simulink model "can2_mcu_power_unpack"  (R2026b)
settings: Solver=VariableStepAuto
libraries: simulink x1, svdutilitieslib x1
settings Model: Creator=aomar  LastModifiedBy=aomar

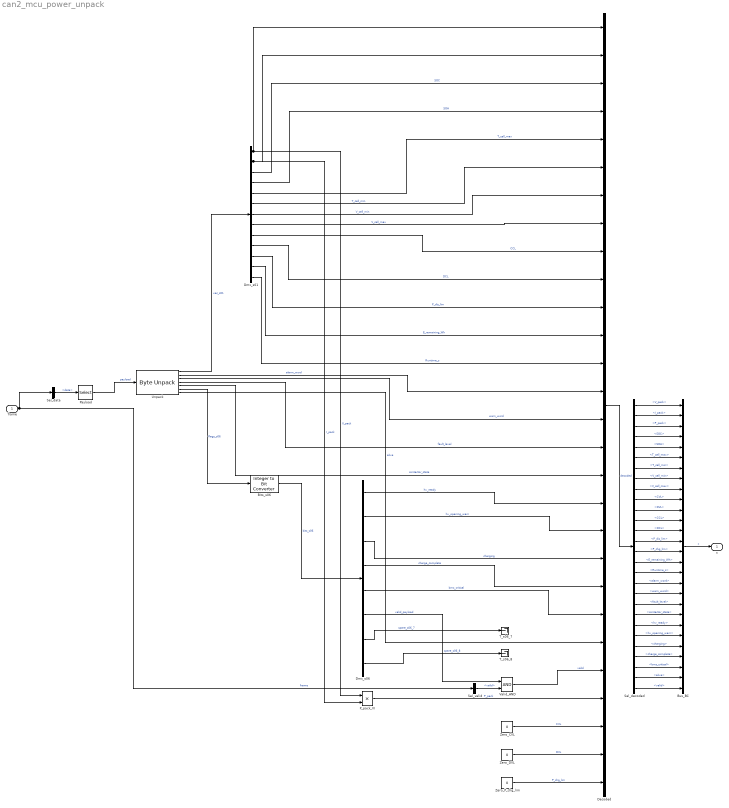
== system can2_mcu_power_unpack ==
  frame : Inport  OutDataTypeStr=Bus: Bus_CanFrame64
  Bits_s06 : simulink/Logic and Bit Operations/Integer to Bit Converter  nbits=8  signedInputValues=Unsigned  bitOrder=LSB first  outDtype=boolean
      settings: LibrarySourceBlock=|
      | commutil2/Integer to Bit
      | Converter
  Bus_BC : BusCreator  Inputs=28  OutDataTypeStr=Bus: Bus_BmsStatus  NonVirtualBus=on
      settings: InheritFromInputs=off
  Decoded : BusCreator  Inputs=28
  Dmx_s01 : Demux  Outputs=13
  Dmx_s06 : Demux  Outputs=8
  P_pack_VI : Product
  Payload : Selector  InputPortWidth=64  IndexOptions=Index vector (dialog)  Indices=1:64  OutputSizes=1
  Sel_data : BusSelector  OutputSignals=data
  Sel_decoded : BusSelector  OutputSignals=V_pack,I_pack,P_pack,SOC,SOH,T_cell_max,T_cell_min,V_cell_min,V_cell_max,CVL,DVL,CCL,DCL,P_dis_lim,P_chg_lim,E_remaining_Wh,Runtime_s,alarm_word,warn_word,fault_level,contactor_state,hv_ready,hv_opening_warn,charging,charge_complete,bms_critical,alive,valid
  Sel_valid : BusSelector  OutputSignals=valid
  T_s06_7 : Terminator
  T_s06_8 : Terminator
  Unpack : svdutilitieslib/Byte Unpack  dimensions={13,1,1,1,1,1,1}  datatypes={'single','uint32','uint32','uint8','uint8','uint8','uint8'}  byteAlign=1  blockPlatform=arduinoert
      settings: LibrarySourceBlock=mcblib/Signal Management/Byte Unpack
  Valid_AND : Logic  AllPortsSameDT=off  OutDataTypeStr=boolean
  Zero_CVL : Constant  Value=0  OutDataTypeStr=single  SampleTime=-1
  Zero_DVL : Constant  Value=0  OutDataTypeStr=single  SampleTime=-1
  Zero_P_chg_lim : Constant  Value=0  OutDataTypeStr=single  SampleTime=-1
  x : Outport  OutDataTypeStr=Bus: Bus_BmsStatus
  wires:
  frame/1 -> Sel_valid/1, Sel_data/1  "frame"
  Sel_data/1 -> Payload/1  "<data>"
  Payload/1 -> Unpack/1  "payload"
  Unpack/1 -> Dmx_s01/1  "vec_s01"
  Unpack/2 -> Decoded/14  "alarm_word"
  Unpack/3 -> Decoded/15  "warn_word"
  Unpack/4 -> Decoded/16  "fault_level"
  Unpack/5 -> Decoded/17  "contactor_state"
  Unpack/6 -> Bits_s06/1  "flags_s06"
  Unpack/7 -> Decoded/23  "alive"
  Dmx_s01/1 -> P_pack_VI/1, Decoded/1  "V_pack"
  Dmx_s01/2 -> P_pack_VI/2, Decoded/2  "I_pack"
  Dmx_s01/3 -> Decoded/3  "SOC"
  Dmx_s01/4 -> Decoded/4  "SOH"
  Dmx_s01/5 -> Decoded/5  "T_cell_max"
  Dmx_s01/6 -> Decoded/6  "T_cell_min"
  Dmx_s01/7 -> Decoded/7  "V_cell_min"
  Dmx_s01/8 -> Decoded/8  "V_cell_max"
  Dmx_s01/9 -> Decoded/9  "CCL"
  Dmx_s01/10 -> Decoded/10  "DCL"
  Dmx_s01/11 -> Decoded/11  "P_dis_lim"
  Dmx_s01/12 -> Decoded/12  "E_remaining_Wh"
  Dmx_s01/13 -> Decoded/13  "Runtime_s"
  Bits_s06/1 -> Dmx_s06/1  "bits_s06"
  Dmx_s06/1 -> Decoded/18  "hv_ready"
  Dmx_s06/2 -> Decoded/19  "hv_opening_warn"
  Dmx_s06/3 -> Decoded/20  "charging"
  Dmx_s06/4 -> Decoded/21  "charge_complete"
  Dmx_s06/5 -> Decoded/22  "bms_critical"
  Dmx_s06/6 -> Valid_AND/1  "valid_payload"
  Dmx_s06/7 -> T_s06_7/1  "spare_s06_7"
  Dmx_s06/8 -> T_s06_8/1  "spare_s06_8"
  P_pack_VI/1 -> Decoded/25  "P_pack"
  Sel_valid/1 -> Valid_AND/2  "<valid>"
  Valid_AND/1 -> Decoded/24  "valid"
  Zero_CVL/1 -> Decoded/26  "CVL"
  Zero_DVL/1 -> Decoded/27  "DVL"
  Zero_P_chg_lim/1 -> Decoded/28  "P_chg_lim"
  Decoded/1 -> Sel_decoded/1  "decoded"
  Sel_decoded/1 -> Bus_BC/1  "<V_pack>"
  Sel_decoded/2 -> Bus_BC/2  "<I_pack>"
  Sel_decoded/3 -> Bus_BC/3  "<P_pack>"
  Sel_decoded/4 -> Bus_BC/4  "<SOC>"
  Sel_decoded/5 -> Bus_BC/5  "<SOH>"
  Sel_decoded/6 -> Bus_BC/6  "<T_cell_max>"
  Sel_decoded/7 -> Bus_BC/7  "<T_cell_min>"
  Sel_decoded/8 -> Bus_BC/8  "<V_cell_min>"
  Sel_decoded/9 -> Bus_BC/9  "<V_cell_max>"
  Sel_decoded/10 -> Bus_BC/10  "<CVL>"
  Sel_decoded/11 -> Bus_BC/11  "<DVL>"
  Sel_decoded/12 -> Bus_BC/12  "<CCL>"
  Sel_decoded/13 -> Bus_BC/13  "<DCL>"
  Sel_decoded/14 -> Bus_BC/14  "<P_dis_lim>"
  Sel_decoded/15 -> Bus_BC/15  "<P_chg_lim>"
  Sel_decoded/16 -> Bus_BC/16  "<E_remaining_Wh>"
  Sel_decoded/17 -> Bus_BC/17  "<Runtime_s>"
  Sel_decoded/18 -> Bus_BC/18  "<alarm_word>"
  Sel_decoded/19 -> Bus_BC/19  "<warn_word>"
  Sel_decoded/20 -> Bus_BC/20  "<fault_level>"
  Sel_decoded/21 -> Bus_BC/21  "<contactor_state>"
  Sel_decoded/22 -> Bus_BC/22  "<hv_ready>"
  Sel_decoded/23 -> Bus_BC/23  "<hv_opening_warn>"
  Sel_decoded/24 -> Bus_BC/24  "<charging>"
  Sel_decoded/25 -> Bus_BC/25  "<charge_complete>"
  Sel_decoded/26 -> Bus_BC/26  "<bms_critical>"
  Sel_decoded/27 -> Bus_BC/27  "<alive>"
  Sel_decoded/28 -> Bus_BC/28  "<valid>"
  Bus_BC/1 -> x/1  "x"
